simulink model "six_pulse_dstack_based_rectifier"  (R2026a)
settings: Solver=ode23tb  StopTime=simlength  FixedStep=Ts  MaxStep=Tc  EnableMultiTasking=on
values from neighbouring files (symbols this model uses):
  Csnubber = 0.1e-6    (= 1e-07)    [init_model.m]
  LFu_dc = 1.2e-3    (= 0.0012)    [init_model.m]
  Rgrading = 2.4e6    (= 2400000)    [init_model.m]
  RLFu_dc = 2e-4    (= 0.0002)    [init_model.m]
  Rsnubber = 1000    [init_model.m]
  Tc = Tcontrol_rect/4000    (= 5e-08)    [init_model.m]
  Tcontrol_rect = tPWM_RECT    (= 0.0002)    [init_model.m]
  Vnom_ac_adc = 400/sqrt(3)*sqrt(2)    [init_model.m]
  w_grid = f_grid*2*pi    (= 314.159265359)    [init_model.m]
undefined symbols (not defined in the file or in its folder): magnitude, rms
libraries: fl_lib x179, nesl_utility x129, diode_rr_lib x36, ee_lib x2
(part 1 of 5)
settings Model: Creator=LTNBDA  LastModifiedBy=d.bagnara
settings SolverCC: ZeroCrossControl=EnableAll  ZeroCrossAlgorithm=Adaptive  SolverResetMethod=Robust
settings DataIOCC: MaxDataPoints=1  SignalLoggingSaveFormat=ModelDataLogs
settings OptimizationCC: InitFltsAndDblsToZero=on  EfficientMapNaN2IntZero=off
settings DebuggingCC: SaveWithParameterizedLinksMsg=none  SignalResolutionControl=TryResolveAllWithWarning  MultiTaskDSMMsg=warning  MultiTaskCondExecSysMsg=none
settings HardwareCC: ProdBitPerLong=64.0  ProdHWDeviceType=Generic->64-bit Embedded Processor (LP64)  TargetBitPerPointer=64.0  TargetBitPerSizeT=64.0  TargetBitPerPtrDiffT=64.0  TargetLongLongMode=on  TargetIntDivRoundTo=Zero  TargetEndianess=LittleEndian  TargetWordSize=64.0  TargetHWDeviceType=MATLAB Host  ProdEqTarget=off
settings SFSimCC: SimCustomHeaderCode=|
  | #include "math_f.h"
  | #include "mavgflt.h"
  | #include "mavgflt_simulink.h"
  | #include "bemf_obsv.h"
  | #include "bemf_obsv_simulink.h"
  | #include "bemf_obsv_load_est.h"
  | #include "bemf_obsv_load_est_simulink.h"
  | #include "dqvector_pi.h"
  | #include "dqvector_pi_simulink.h"
  | #include "sv_pwm_simulink.h"
  | #include "sv_pwm.h"
  | #include "six_pulse_rect.h"
  | #include "twelve_pulse_rect.h"
  | #include "first_harmonic_tracker.h"
  | #include "first_harmonic_tracker_simulink.h"
  | #include "dqpll_thyr.h"
  | #include "dqpll_thyr_simulink.h"
  | #include "dqpll_grid.h"
  | #include "dqpll_grid_simulink.h"
settings SFSimCC: SimUserSources=|
  | "mavgflt_simulink.c"
  | "mavgflt.c"
  | "bemf_obsv_simulink.c"
  | "bemf_obsv.c"
  | "bemf_obsv_load_est_simulink.c"
  | "bemf_obsv_load_est.c"
  | "dqvector_pi.c"
  | "dqvector_pi_simulink.c"
  | "sv_pwm_simulink.c"
  | "sv_pwm.c"
  | "six_pulse_rect.c"
  | "twelve_pulse_rect.c"
  | "first_harmonic_tracker_simulink.c"
  | "first_harmonic_tracker.c"
  | "dqpll_thyr_simulink.c"
  | "dqpll_thyr.c"
  | "dqpll_grid_simulink.c"
  | "dqpll_grid.c"
settings SFSimCC: SimUserIncludeDirs=|
  | include
  | src
settings CodeAppCC: MaxIdLength=128.0
settings GRTTargetCC: CombineOutputUpdateFcns=off  GRTInterface=on
settings SimscapeCC: SimscapeNormalizeSystem=off  SimscapeNominalValues="[{\"value\":\"1\",\"unit\":\"A\"},{\"value\":\"1\",\"unit\":\"bar\"},{\"value\":\"1\",\"unit\":\"cm^2\"},{\"value\":\"1\",\"unit\":\"cm^3/s\"},{\"value\":\"1\",\"unit\":\"kJ/kg\"},{\"value\":\"1\",\"unit\":\"kW\"},{\"value\":\"1\",\"unit\":\"l\"},{\"value\":\"1\",\"unit\":\"N\"},{\"value\":\"1\",\"unit\":\"N*m\"},{\"value\":\"1\",\"unit\":\"V\"}]"  SimscapeLogType=none  SimscapeLogDataHistory=5000.0

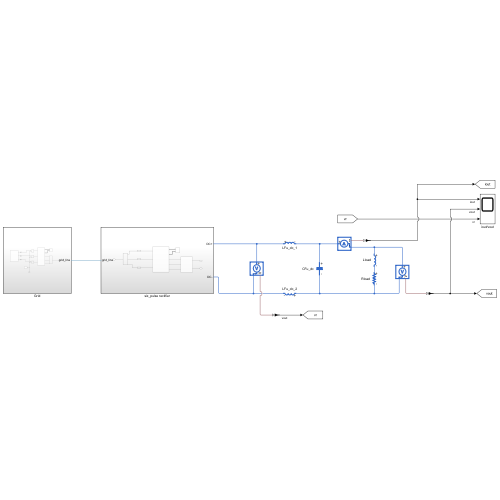
[thumbnail: Simulink's stored preview of the top-level diagram]
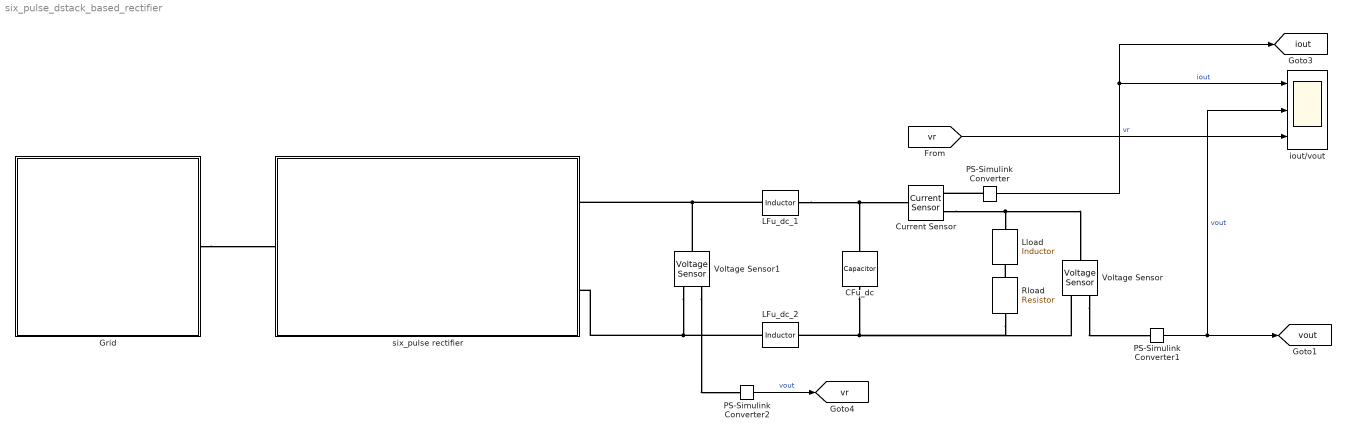
== system six_pulse_dstack_based_rectifier ==
  CFu_dc : fl_lib/Electrical/Electrical Elements/Capacitor  c=CFu_dc F  r=RCFu_dc Ohm  g=0 1/Ohm  i_specify=off  i_priority=None  i=0 A  i_nominal_specify=off  i_nominal_value=1  i_nominal_unit=A  v_specify=off  v_priority=None  v=0 V  v_nominal_specify=off  v_nominal_value=1  v_nominal_unit=V  vc_specify=off  vc_priority=High  vc=0 V  vc_nominal_specify=off  vc_nominal_value=1  vc_nominal_unit=V
  Current Sensor : fl_lib/Electrical/Electrical Sensors/Current Sensor
  Grid : Subsystem
  LFu_dc_1 : fl_lib/Electrical/Electrical Elements/Inductor  l=LFu_dc/2 H  r=RLFu_dc/2 Ohm  g=1e-9 1/Ohm  i_specify=off  i_priority=None  i=0 A  i_nominal_specify=off  i_nominal_value=1  i_nominal_unit=A  v_specify=off  v_priority=None  v=0 V  v_nominal_specify=off  v_nominal_value=1  v_nominal_unit=V  i_L_specify=off  i_L_priority=High  i_L=0 A  i_L_nominal_specify=off  i_L_nominal_value=1  i_L_nominal_unit=A
  LFu_dc_2 : fl_lib/Electrical/Electrical Elements/Inductor  l=LFu_dc/2 H  r=RLFu_dc/2 Ohm  g=1e-9 1/Ohm  i_specify=off  i_priority=None  i=0 A  i_nominal_specify=off  i_nominal_value=1  i_nominal_unit=A  v_specify=off  v_priority=None  v=0 V  v_nominal_specify=off  v_nominal_value=1  v_nominal_unit=V  i_L_specify=off  i_L_priority=High  i_L=0 A  i_L_nominal_specify=off  i_L_nominal_value=1  i_L_nominal_unit=A
  Lload : fl_lib/Electrical/Electrical Elements/Inductor  l=Lload H  r=0 Ohm  g=1e-9 1/Ohm  i_specify=off  i_priority=None  i=0 A  i_nominal_specify=off  i_nominal_value=1  i_nominal_unit=A  v_specify=off  v_priority=None  v=0 V  v_nominal_specify=off  v_nominal_value=1  v_nominal_unit=V  i_L_specify=off  i_L_priority=High  i_L=0 A  i_L_nominal_specify=off  i_L_nominal_value=1  i_L_nominal_unit=A
  PS-Simulink Converter : nesl_utility/PS-Simulink Converter  PhysicalDomain=network_engine_domain  SubClassName=ps_output  LeftPortType=input  RightPortType=output  PseudoPeriodic=off  Frequencies=[]  VectorFormat=1-D array  Unit=A  AffineConversion=off
  PS-Simulink Converter1 : nesl_utility/PS-Simulink Converter  PhysicalDomain=network_engine_domain  SubClassName=ps_output  LeftPortType=input  RightPortType=output  PseudoPeriodic=off  Frequencies=[]  VectorFormat=1-D array  Unit=V  AffineConversion=on
  PS-Simulink Converter2 : nesl_utility/PS-Simulink Converter  PhysicalDomain=network_engine_domain  SubClassName=ps_output  LeftPortType=input  RightPortType=output  PseudoPeriodic=off  Frequencies=[]  VectorFormat=1-D array  Unit=V  AffineConversion=on
  Rload : fl_lib/Electrical/Electrical Elements/Resistor  R=(13.8e3*1.35)^2/1e6 Ohm  i_specify=off  i_priority=None  i=0 A  i_nominal_specify=off  i_nominal_value=1  i_nominal_unit=A  v_specify=off  v_priority=None  v=0 V  v_nominal_specify=off  v_nominal_value=1  v_nominal_unit=V
  Voltage Sensor : fl_lib/Electrical/Electrical Sensors/Voltage Sensor
  Voltage Sensor1 : fl_lib/Electrical/Electrical Sensors/Voltage Sensor
  iout/vout : Scope  NumInputPorts=3
      settings: ActiveDisplayYMinimum=54.4311221075266  ActiveDisplayYMaximum=54.825714064717985  DataLoggingVariableName=ScopeData10
  six_pulse rectifier : Subsystem
  tag scope: iout=global, vout=global, vr=global
  wires:
  PS-Simulink Converter/1 -> [iout], iout/vout/1  "iout"
  PS-Simulink Converter1/1 -> [vout], iout/vout/2  "vout"
  PS-Simulink Converter2/1 -> [vr]  "vout"
  [vr] -> iout/vout/3  "vr"
  connections:
  LFu_dc_1/RConn1 -- CFu_dc/LConn1 -- Current Sensor/LConn1
  CFu_dc/RConn1 -- Voltage Sensor/RConn2 -- Rload/RConn1 -- LFu_dc_2/LConn1
  LFu_dc_2/RConn1 -- Voltage Sensor1/RConn2 -- six_pulse rectifier/RConn2
  LFu_dc_1/LConn1 -- six_pulse rectifier/RConn1 -- Voltage Sensor1/LConn1
  Rload/LConn1 -- Lload/RConn1
  PS-Simulink Converter/LConn1 -- Current Sensor/RConn1
  Current Sensor/RConn2 -- Voltage Sensor/LConn1 -- Lload/LConn1
  Voltage Sensor/RConn1 -- PS-Simulink Converter1/LConn1
  Voltage Sensor1/RConn1 -- PS-Simulink Converter2/LConn1
  Grid/RConn1 -- six_pulse rectifier/LConn1

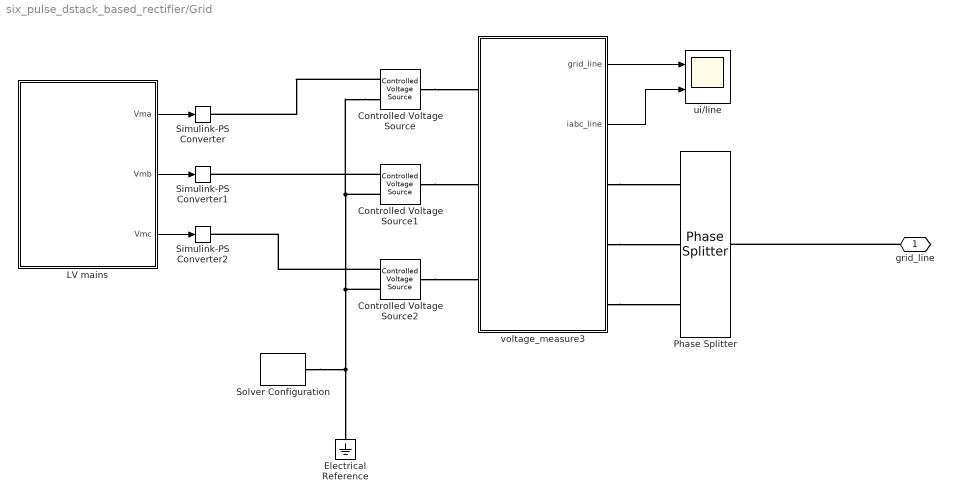
== system six_pulse_dstack_based_rectifier/Grid ==
  Controlled Voltage Source : fl_lib/Electrical/Electrical Sources/Controlled Voltage Source
  Controlled Voltage Source1 : fl_lib/Electrical/Electrical Sources/Controlled Voltage Source
  Controlled Voltage Source2 : fl_lib/Electrical/Electrical Sources/Controlled Voltage Source
  Electrical Reference : fl_lib/Electrical/Electrical Elements/Electrical Reference
  LV mains : Subsystem
  Phase Splitter : ee_lib/Connectors & References/Phase Splitter
  Simulink-PS Converter : nesl_utility/Simulink-PS Converter  PhysicalDomain=network_engine_domain  SubClassName=ps_input  LeftPortType=input  RightPortType=output  PseudoPeriodic=off  Frequencies=[]  NoiseDistribution=none  NoiseParameters=[]  Unit=V  AffineConversion=on  FilteringAndDerivatives=provide  SimscapeFilterOrder=1  InputFilterTimeConstant=0.001  UdotUserProvided=0
  Simulink-PS Converter1 : nesl_utility/Simulink-PS Converter  PhysicalDomain=network_engine_domain  SubClassName=ps_input  LeftPortType=input  RightPortType=output  PseudoPeriodic=off  Frequencies=[]  NoiseDistribution=none  NoiseParameters=[]  Unit=V  AffineConversion=on  FilteringAndDerivatives=provide  SimscapeFilterOrder=1  InputFilterTimeConstant=0.001  UdotUserProvided=0
  Simulink-PS Converter2 : nesl_utility/Simulink-PS Converter  PhysicalDomain=network_engine_domain  SubClassName=ps_input  LeftPortType=input  RightPortType=output  PseudoPeriodic=off  Frequencies=[]  NoiseDistribution=none  NoiseParameters=[]  Unit=V  AffineConversion=on  FilteringAndDerivatives=provide  SimscapeFilterOrder=1  InputFilterTimeConstant=0.001  UdotUserProvided=0
  Solver Configuration : nesl_utility/Solver Configuration  PhysicalDomain=network_engine_domain  SubClassName=solver  LeftPortType=input  RightPortType=generic  Tones=[]  Harmonics=[]  SimulateNoise=off  Profile=off  UseLocalSampling=off  EnableSwitchedLinearOptims=on  FrequencyDomain=off  UseCCode=off  RelTol=0.001  AbsTol=1e-06  MinStep=1e-09  ToWorkspace=off  RevertToSquareIcSolve=off  NumHomotopyIterations=100  PhasorMode=off  PhasorModeNumHarmonics=1  ConsistencySolver=NEWTON_FTOL  CanonicalOrdering=UNORDERED  OptimizeIntermediates=UNOPTIMIZED  IndexReductionMethod=DerivativeReplacement  DoDC=on  ResidualTolerance=1e-4  ConsistencyTolSource=GLOBAL  ConsistencyAbsTol=0.001  ConsistencyRelTol=0.001  ConsistencyTolFactor=0.001  UseLocalSolver=on  LocalSolverChoice=NE_TRAPEZOIDAL_ADVANCER  ResolveIndetEquations=on  FunctionEvalNumThread=1  LocalSolverSampleTime=Tc  DoFixedCost=on  MaxNonlinIter=5  MaxModeIter=2  ComputeImpulses=off  ImpulseIterations=2  LinearAlgebra=auto  LinearAlgebraNumThread=0  EquationFormulation=NE_TIME_EF  DelaysMemoryBudget=1024  AutomaticFiltering=on  FilteringTimeConstant=0.001  PartitionStorageMethod=AS_NEEDED  PartitionMemoryBudget=1024  PartitionMethod=ROBUST  MultibodyUseLocalSolver=off  MultibodyLocalSolverChoice=ODE1  MultibodyLocalSolverSampleTime=0.001
  ui/line : Scope  NumInputPorts=2
      settings: SampleTime=Tcontrol_rect  ActiveDisplayYMinimum=-1.25  ActiveDisplayYMaximum=1.25
  voltage_measure3 : Subsystem
  grid_line : PMIOPort  Side=Right
  wires:
  voltage_measure3/2(iabc_line) -> ui/line/2
  LV mains/1(Vma) -> Simulink-PS Converter/1
  LV mains/3(Vmc) -> Simulink-PS Converter2/1
  LV mains/2(Vmb) -> Simulink-PS Converter1/1
  voltage_measure3/1(grid_line) -> ui/line/1
  connections:
  Controlled Voltage Source1/LConn1 -- voltage_measure3/LConn2
  grid_line/RConn1 -- Phase Splitter/LConn1
  Controlled Voltage Source/RConn1 -- Simulink-PS Converter/RConn1
  Controlled Voltage Source/RConn2 -- Controlled Voltage Source1/RConn2 -- Controlled Voltage Source2/RConn2 -- Solver Configuration/RConn1 -- Electrical Reference/LConn1
  voltage_measure3/RConn2 -- Phase Splitter/RConn2
  Controlled Voltage Source2/LConn1 -- voltage_measure3/LConn3
  voltage_measure3/RConn3 -- Phase Splitter/RConn3
  Controlled Voltage Source1/RConn1 -- Simulink-PS Converter1/RConn1
  Controlled Voltage Source2/RConn1 -- Simulink-PS Converter2/RConn1
  Controlled Voltage Source/LConn1 -- voltage_measure3/LConn1
  voltage_measure3/RConn1 -- Phase Splitter/RConn1

== system six_pulse_dstack_based_rectifier/six_pulse rectifier ==
  BR2 : Subsystem
  Lgrid_U : fl_lib/Electrical/Electrical Elements/Inductor  l=31e-3 H  r=0 Ohm  g=1e-9 1/Ohm  i_specify=off  i_priority=None  i=0 A  i_nominal_specify=off  i_nominal_value=1  i_nominal_unit=A  v_specify=off  v_priority=None  v=0 V  v_nominal_specify=off  v_nominal_value=1  v_nominal_unit=V  i_L_specify=off  i_L_priority=High  i_L=0 A  i_L_nominal_specify=off  i_L_nominal_value=1  i_L_nominal_unit=A
  Lgrid_V : fl_lib/Electrical/Electrical Elements/Inductor  l=31e-3 H  r=0 Ohm  g=1e-9 1/Ohm  i_specify=off  i_priority=None  i=0 A  i_nominal_specify=off  i_nominal_value=1  i_nominal_unit=A  v_specify=off  v_priority=None  v=0 V  v_nominal_specify=off  v_nominal_value=1  v_nominal_unit=V  i_L_specify=off  i_L_priority=High  i_L=0 A  i_L_nominal_specify=off  i_L_nominal_value=1  i_L_nominal_unit=A
  Lgrid_W : fl_lib/Electrical/Electrical Elements/Inductor  l=31e-3 H  r=0 Ohm  g=1e-9 1/Ohm  i_specify=off  i_priority=None  i=0 A  i_nominal_specify=off  i_nominal_value=1  i_nominal_unit=A  v_specify=off  v_priority=None  v=0 V  v_nominal_specify=off  v_nominal_value=1  v_nominal_unit=V  i_L_specify=off  i_L_priority=High  i_L=0 A  i_L_nominal_specify=off  i_L_nominal_value=1  i_L_nominal_unit=A
  Phase Splitter2 : ee_lib/Connectors & References/Phase Splitter
  ui/grid : Scope  NumInputPorts=2
      settings: ActiveDisplayYMinimum=-46.896074870279  ActiveDisplayYMaximum=64.47147383027982
  voltage_measure2 : Subsystem
  DC+ : PMIOPort  Side=Right
  grid_line : PMIOPort  Port=2  Side=Left
  DC- : PMIOPort  Port=3  Side=Right
  wires:
  voltage_measure2/1(vabc_grid) -> ui/grid/1
  voltage_measure2/2(iabc_grid) -> ui/grid/2
  connections:
  voltage_measure2/RConn1 -- BR2/RConn1
  grid_line/RConn1 -- Phase Splitter2/LConn1
  BR2/LConn2 -- DC-/RConn1
  voltage_measure2/RConn3 -- BR2/RConn3
  Lgrid_U/RConn1 -- voltage_measure2/LConn1
  voltage_measure2/RConn2 -- BR2/RConn2
  BR2/LConn1 -- DC+/RConn1
  Phase Splitter2/RConn1 -- Lgrid_U/LConn1
  Lgrid_V/RConn1 -- voltage_measure2/LConn2
  Lgrid_V/LConn1 -- Phase Splitter2/RConn2
  Lgrid_W/LConn1 -- Phase Splitter2/RConn3
  Lgrid_W/RConn1 -- voltage_measure2/LConn3

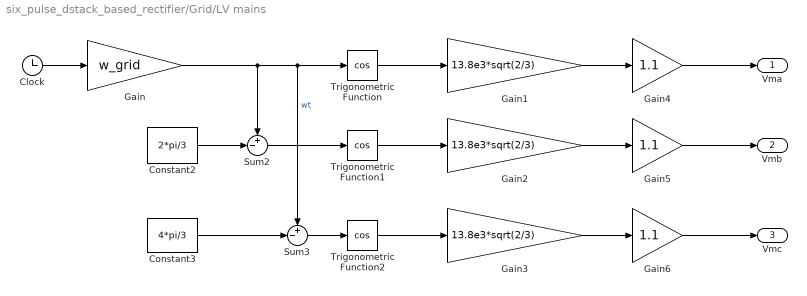
== system six_pulse_dstack_based_rectifier/Grid/LV mains ==
  Clock : Clock
  Constant2 : Constant  Value=2*pi/3
  Constant3 : Constant  Value=4*pi/3
  Gain : Gain  Gain=w_grid
  Gain1 : Gain  Gain=13.8e3*sqrt(2/3)
  Gain2 : Gain  Gain=13.8e3*sqrt(2/3)
  Gain3 : Gain  Gain=13.8e3*sqrt(2/3)
  Gain4 : Gain  Gain=1.1
  Gain5 : Gain  Gain=1.1
  Gain6 : Gain  Gain=1.1
  Sum2 : Sum  Inputs=+-|
  Sum3 : Sum  Inputs=+-|
  Trigonometric Function : Trigonometry  Operator=cos
  Trigonometric Function1 : Trigonometry  Operator=cos
  Trigonometric Function2 : Trigonometry  Operator=cos
  Vma : Outport
  Vmb : Outport  Port=2
  Vmc : Outport  Port=3
  wires:
  Trigonometric Function/1 -> Gain1/1
  Constant2/1 -> Sum2/2
  Sum2/1 -> Trigonometric Function1/1
  Constant3/1 -> Sum3/2
  Sum3/1 -> Trigonometric Function2/1
  Clock/1 -> Gain/1
  Gain/1 -> Sum3/1, Trigonometric Function/1, Sum2/1  "wt"
  Trigonometric Function1/1 -> Gain2/1
  Trigonometric Function2/1 -> Gain3/1
  Gain1/1 -> Gain4/1
  Gain2/1 -> Gain5/1
  Gain3/1 -> Gain6/1
  Gain4/1 -> Vma/1
  Gain5/1 -> Vmb/1
  Gain6/1 -> Vmc/1

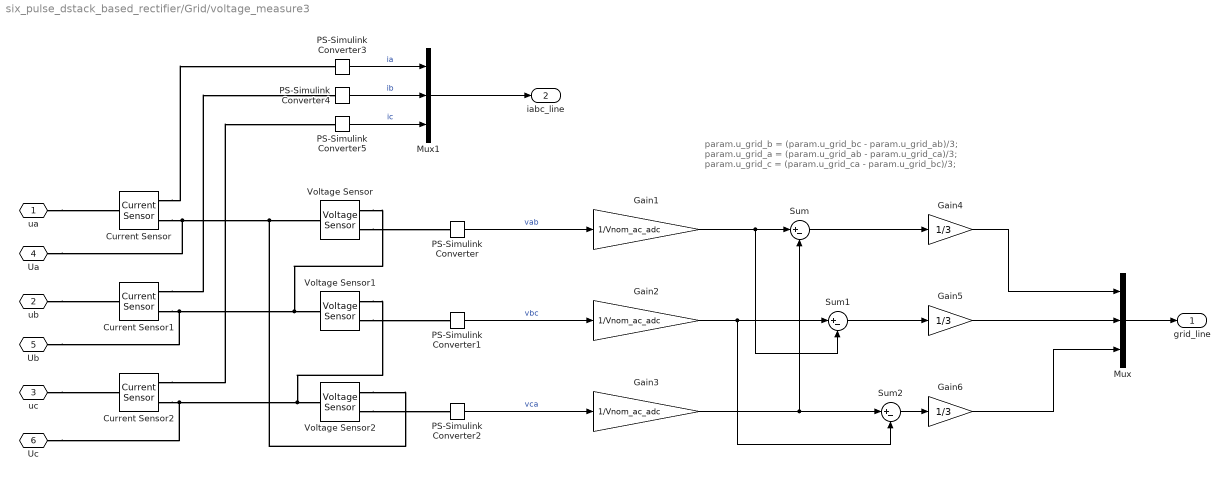
== system six_pulse_dstack_based_rectifier/Grid/voltage_measure3 ==
  note: param.u_grid_b = (param.u_grid_bc - param.u_grid_ab)/3;
      | 	param.u_grid_a = (param.u_grid_ab - param.u_grid_ca)/3;
      | 	param.u_grid_c = (param.u_grid_ca - param.u_grid_bc)/3;
  Current Sensor : fl_lib/Electrical/Electrical Sensors/Current Sensor
  Current Sensor1 : fl_lib/Electrical/Electrical Sensors/Current Sensor
  Current Sensor2 : fl_lib/Electrical/Electrical Sensors/Current Sensor
  Gain1 : Gain  Gain=1/Vnom_ac_adc
  Gain2 : Gain  Gain=1/Vnom_ac_adc
  Gain3 : Gain  Gain=1/Vnom_ac_adc
  Gain4 : Gain  Gain=1/3
  Gain5 : Gain  Gain=1/3
  Gain6 : Gain  Gain=1/3
  Mux : Mux  Inputs=3
  Mux1 : Mux  Inputs=3
  PS-Simulink Converter : nesl_utility/PS-Simulink Converter  PhysicalDomain=network_engine_domain  SubClassName=ps_output  LeftPortType=input  RightPortType=output  PseudoPeriodic=off  Frequencies=[]  VectorFormat=1-D array  Unit=inherit  AffineConversion=off
  PS-Simulink Converter1 : nesl_utility/PS-Simulink Converter  PhysicalDomain=network_engine_domain  SubClassName=ps_output  LeftPortType=input  RightPortType=output  PseudoPeriodic=off  Frequencies=[]  VectorFormat=1-D array  Unit=inherit  AffineConversion=off
  PS-Simulink Converter2 : nesl_utility/PS-Simulink Converter  PhysicalDomain=network_engine_domain  SubClassName=ps_output  LeftPortType=input  RightPortType=output  PseudoPeriodic=off  Frequencies=[]  VectorFormat=1-D array  Unit=inherit  AffineConversion=off
  PS-Simulink Converter3 : nesl_utility/PS-Simulink Converter  PhysicalDomain=network_engine_domain  SubClassName=ps_output  LeftPortType=input  RightPortType=output  PseudoPeriodic=off  Frequencies=[]  VectorFormat=1-D array  Unit=A  AffineConversion=off
  PS-Simulink Converter4 : nesl_utility/PS-Simulink Converter  PhysicalDomain=network_engine_domain  SubClassName=ps_output  LeftPortType=input  RightPortType=output  PseudoPeriodic=off  Frequencies=[]  VectorFormat=1-D array  Unit=A  AffineConversion=off
  PS-Simulink Converter5 : nesl_utility/PS-Simulink Converter  PhysicalDomain=network_engine_domain  SubClassName=ps_output  LeftPortType=input  RightPortType=output  PseudoPeriodic=off  Frequencies=[]  VectorFormat=1-D array  Unit=A  AffineConversion=off
  Sum : Sum  Inputs=|+-
  Sum1 : Sum  Inputs=|+-
  Sum2 : Sum  Inputs=|+-
  Voltage Sensor : fl_lib/Electrical/Electrical Sensors/Voltage Sensor
  Voltage Sensor1 : fl_lib/Electrical/Electrical Sensors/Voltage Sensor
  Voltage Sensor2 : fl_lib/Electrical/Electrical Sensors/Voltage Sensor
  ua : PMIOPort  Side=Left
  ub : PMIOPort  Port=2  Side=Left
  uc : PMIOPort  Port=3  Side=Left
  Ua : PMIOPort  Port=4  Side=Right
  Ub : PMIOPort  Port=5  Side=Right
  Uc : PMIOPort  Port=6  Side=Right
  grid_line : Outport
  iabc_line : Outport  Port=2
  wires:
  PS-Simulink Converter5/1 -> Mux1/3  "ic"
  PS-Simulink Converter3/1 -> Mux1/1  "ia"
  PS-Simulink Converter4/1 -> Mux1/2  "ib"
  Mux1/1 -> iabc_line/1
  Gain6/1 -> Mux/3
  Gain5/1 -> Mux/2
  Gain4/1 -> Mux/1
  Gain2/1 -> Sum1/1, Sum2/2
  Sum2/1 -> Gain6/1
  Sum1/1 -> Gain5/1
  Sum/1 -> Gain4/1
  Gain3/1 -> Sum/2, Sum2/1
  Gain1/1 -> Sum/1, Sum1/2
  Mux/1 -> grid_line/1
  PS-Simulink Converter/1 -> Gain1/1  "vab"
  PS-Simulink Converter2/1 -> Gain3/1  "vca"
  PS-Simulink Converter1/1 -> Gain2/1  "vbc"
  connections:
  Current Sensor2/RConn1 -- PS-Simulink Converter5/LConn1
  Current Sensor1/RConn1 -- PS-Simulink Converter4/LConn1
  Current Sensor/RConn1 -- PS-Simulink Converter3/LConn1
  uc/RConn1 -- Current Sensor2/LConn1
  ub/RConn1 -- Current Sensor1/LConn1
  ua/RConn1 -- Current Sensor/LConn1
  Voltage Sensor1/RConn1 -- PS-Simulink Converter1/LConn1
  Uc/RConn1 -- Current Sensor2/RConn2 -- Voltage Sensor1/RConn2 -- Voltage Sensor2/LConn1
  Voltage Sensor2/RConn1 -- PS-Simulink Converter2/LConn1
  Voltage Sensor/RConn1 -- PS-Simulink Converter/LConn1
  Ua/RConn1 -- Current Sensor/RConn2 -- Voltage Sensor2/RConn2 -- Voltage Sensor/LConn1
  Ub/RConn1 -- Current Sensor1/RConn2 -- Voltage Sensor/RConn2 -- Voltage Sensor1/LConn1

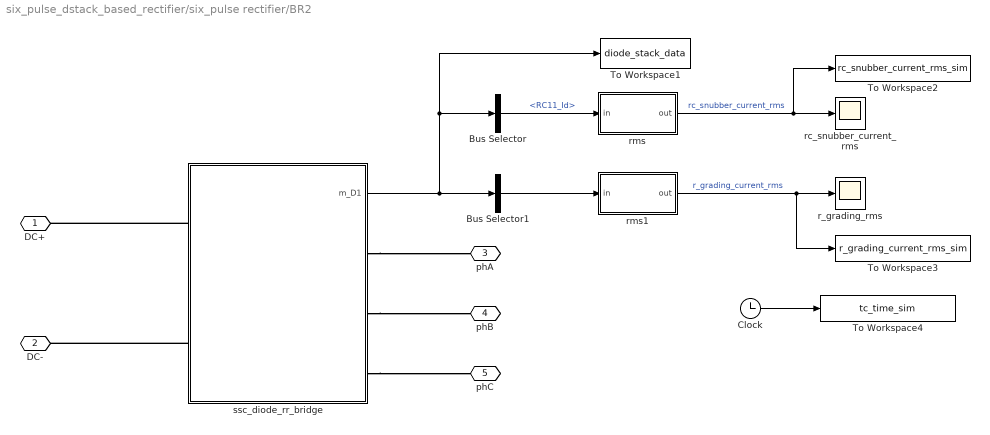
== system six_pulse_dstack_based_rectifier/six_pulse rectifier/BR2 ==
  Bus Selector : BusSelector  OutputSignals=signal1.RC11_Id
  Bus Selector1 : BusSelector  OutputSignals=signal4.Rg11_I  OutputAsBus=on
  Clock : Clock
  To Workspace1 : ToWorkspace  VariableName=diode_stack_data  SaveFormat=Structure With Time  SampleTime=Tc
      settings: MaxDataPoints=Nc
  To Workspace2 : ToWorkspace  VariableName=rc_snubber_current_rms_sim  SaveFormat=Structure With Time  SampleTime=Tc
      settings: MaxDataPoints=Nc
  To Workspace3 : ToWorkspace  VariableName=r_grading_current_rms_sim  SaveFormat=Structure With Time  SampleTime=Tc
      settings: MaxDataPoints=Nc
  To Workspace4 : ToWorkspace  VariableName=tc_time_sim  SaveFormat=Structure With Time  SampleTime=Tc
      settings: MaxDataPoints=Nc
  r_grading_rms : Scope
      settings: ActiveDisplayYMinimum=-0.00012535770795036924  ActiveDisplayYMaximum=0.0011282275135877779
  rc_snubber_current_rms : Scope
      settings: ActiveDisplayYMinimum=-0.017079152210377417  ActiveDisplayYMaximum=0.15371236989339679  DataLoggingVariableName=ScopeData8
  rms : Subsystem
  rms1 : Subsystem
  ssc_diode_rr_bridge : Subsystem  mask{Vf_m=1.12, Ron_m=0.29e-3, Goff_m=1e-5, forward_voltage_threshold_m=50, Vgt_m=1.2, latching_current_m=250e-3, holding_current_m=75e-3, carrier_lifetime_m=100e-6, charge_cross_time_constant_m=190e-6, residual_charge_threshold_m=1e-6, circuit_commutated_turn_off_time_m=800e-6, t_firing_strobe_m=Tcontrol_rect, Rsnubber_m=Rsnubber, Csnubber_m=Csnubber, Rgrading_m=Rgrading}
      mask prompts: Vf_m "Vt [V]"; Ron_m "rt [Ohm]"; Goff_m "Goff [1/Ohm]"; forward_voltage_threshold_m "Voltage Retrigger Threshold [V]"; Vgt_m "Vth [V]"; latching_current_m "latching current [A]"; holding_current_m "holding current [A]"; carrier_lifetime_m "carrier lifetime [s]"; charge_cross_time_constant_m "charge extraction time constant [s]"; residual_charge_threshold_m "residual charge threshold [C]"; circuit_commutated_turn_off_time_m "circuit commutated turn off time [s]"; t_firing_strobe_m "t_firing_strobe [s]"; Rsnubber_m "Rsnubber [Ohm]"; Csnubber_m "Csnubber [F]"; Rgrading_m "Rgrading [Ohm]"
  DC+ : PMIOPort  Side=Left
  DC- : PMIOPort  Port=2  Side=Left
  phA : PMIOPort  Port=3  Side=Right
  phB : PMIOPort  Port=4  Side=Right
  phC : PMIOPort  Port=5  Side=Right
  wires:
  rms/1(out) -> To Workspace2/1, rc_snubber_current_rms/1  "rc_snubber_current_rms"
  ssc_diode_rr_bridge/1(m_D1) -> Bus Selector/1, To Workspace1/1, Bus Selector1/1
  Bus Selector/1 -> rms/1(in)  "<RC11_Id>"
  Bus Selector1/1 -> rms1/1(in)
  rms1/1(out) -> To Workspace3/1, r_grading_rms/1  "r_grading_current_rms"
  Clock/1 -> To Workspace4/1
  connections:
  ssc_diode_rr_bridge/LConn1 -- DC+/RConn1
  ssc_diode_rr_bridge/LConn2 -- DC-/RConn1
  ssc_diode_rr_bridge/RConn1 -- phA/RConn1
  ssc_diode_rr_bridge/RConn2 -- phB/RConn1
  ssc_diode_rr_bridge/RConn3 -- phC/RConn1

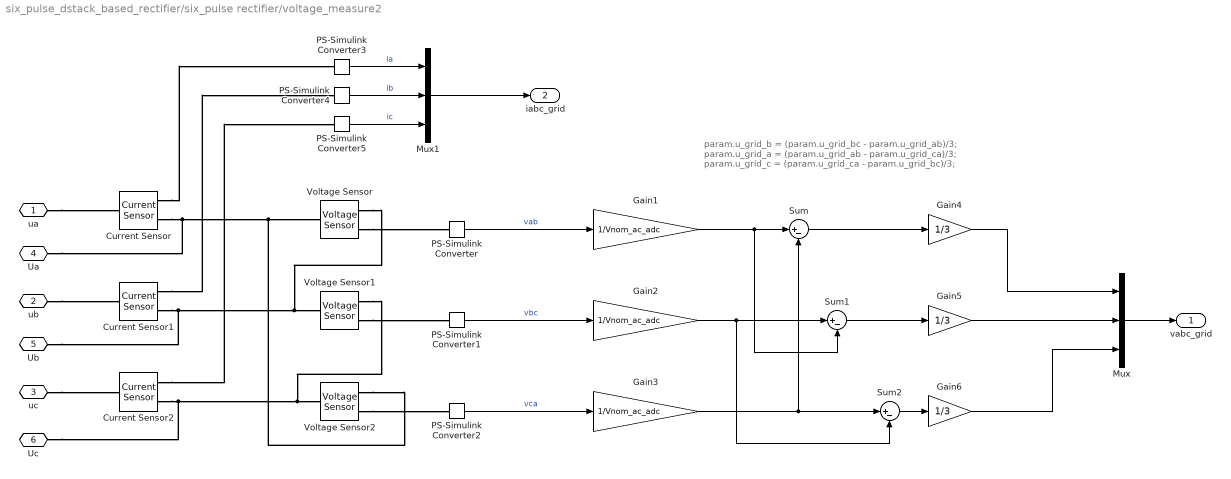
== system six_pulse_dstack_based_rectifier/six_pulse rectifier/voltage_measure2 ==
  note: param.u_grid_b = (param.u_grid_bc - param.u_grid_ab)/3;
      | 	param.u_grid_a = (param.u_grid_ab - param.u_grid_ca)/3;
      | 	param.u_grid_c = (param.u_grid_ca - param.u_grid_bc)/3;
  Current Sensor : fl_lib/Electrical/Electrical Sensors/Current Sensor
  Current Sensor1 : fl_lib/Electrical/Electrical Sensors/Current Sensor
  Current Sensor2 : fl_lib/Electrical/Electrical Sensors/Current Sensor
  Gain1 : Gain  Gain=1/Vnom_ac_adc
  Gain2 : Gain  Gain=1/Vnom_ac_adc
  Gain3 : Gain  Gain=1/Vnom_ac_adc
  Gain4 : Gain  Gain=1/3
  Gain5 : Gain  Gain=1/3
  Gain6 : Gain  Gain=1/3
  Mux : Mux  Inputs=3
  Mux1 : Mux  Inputs=3
  PS-Simulink Converter : nesl_utility/PS-Simulink Converter  PhysicalDomain=network_engine_domain  SubClassName=ps_output  LeftPortType=input  RightPortType=output  PseudoPeriodic=off  Frequencies=[]  VectorFormat=1-D array  Unit=inherit  AffineConversion=off
  PS-Simulink Converter1 : nesl_utility/PS-Simulink Converter  PhysicalDomain=network_engine_domain  SubClassName=ps_output  LeftPortType=input  RightPortType=output  PseudoPeriodic=off  Frequencies=[]  VectorFormat=1-D array  Unit=inherit  AffineConversion=off
  PS-Simulink Converter2 : nesl_utility/PS-Simulink Converter  PhysicalDomain=network_engine_domain  SubClassName=ps_output  LeftPortType=input  RightPortType=output  PseudoPeriodic=off  Frequencies=[]  VectorFormat=1-D array  Unit=inherit  AffineConversion=off
  PS-Simulink Converter3 : nesl_utility/PS-Simulink Converter  PhysicalDomain=network_engine_domain  SubClassName=ps_output  LeftPortType=input  RightPortType=output  PseudoPeriodic=off  Frequencies=[]  VectorFormat=1-D array  Unit=A  AffineConversion=off
  PS-Simulink Converter4 : nesl_utility/PS-Simulink Converter  PhysicalDomain=network_engine_domain  SubClassName=ps_output  LeftPortType=input  RightPortType=output  PseudoPeriodic=off  Frequencies=[]  VectorFormat=1-D array  Unit=A  AffineConversion=off
  PS-Simulink Converter5 : nesl_utility/PS-Simulink Converter  PhysicalDomain=network_engine_domain  SubClassName=ps_output  LeftPortType=input  RightPortType=output  PseudoPeriodic=off  Frequencies=[]  VectorFormat=1-D array  Unit=A  AffineConversion=off
  Sum : Sum  Inputs=|+-
  Sum1 : Sum  Inputs=|+-
  Sum2 : Sum  Inputs=|+-
  Voltage Sensor : fl_lib/Electrical/Electrical Sensors/Voltage Sensor
  Voltage Sensor1 : fl_lib/Electrical/Electrical Sensors/Voltage Sensor
  Voltage Sensor2 : fl_lib/Electrical/Electrical Sensors/Voltage Sensor
  ua : PMIOPort  Side=Left
  ub : PMIOPort  Port=2  Side=Left
  uc : PMIOPort  Port=3  Side=Left
  Ua : PMIOPort  Port=4  Side=Right
  Ub : PMIOPort  Port=5  Side=Right
  Uc : PMIOPort  Port=6  Side=Right
  vabc_grid : Outport
  iabc_grid : Outport  Port=2
  wires:
  PS-Simulink Converter1/1 -> Gain2/1  "vbc"
  PS-Simulink Converter2/1 -> Gain3/1  "vca"
  PS-Simulink Converter/1 -> Gain1/1  "vab"
  Mux/1 -> vabc_grid/1
  Gain1/1 -> Sum1/2, Sum/1
  Gain3/1 -> Sum2/1, Sum/2
  Sum/1 -> Gain4/1
  Sum1/1 -> Gain5/1
  Sum2/1 -> Gain6/1
  Gain2/1 -> Sum2/2, Sum1/1
  Gain4/1 -> Mux/1
  Gain5/1 -> Mux/2
  Gain6/1 -> Mux/3
  Mux1/1 -> iabc_grid/1
  PS-Simulink Converter4/1 -> Mux1/2  "ib"
  PS-Simulink Converter3/1 -> Mux1/1  "ia"
  PS-Simulink Converter5/1 -> Mux1/3  "ic"
  connections:
  Ub/RConn1 -- Current Sensor1/RConn2 -- Voltage Sensor/RConn2 -- Voltage Sensor1/LConn1
  Ua/RConn1 -- Current Sensor/RConn2 -- Voltage Sensor2/RConn2 -- Voltage Sensor/LConn1
  Voltage Sensor/RConn1 -- PS-Simulink Converter/LConn1
  Voltage Sensor2/RConn1 -- PS-Simulink Converter2/LConn1
  Uc/RConn1 -- Current Sensor2/RConn2 -- Voltage Sensor1/RConn2 -- Voltage Sensor2/LConn1
  Voltage Sensor1/RConn1 -- PS-Simulink Converter1/LConn1
  ua/RConn1 -- Current Sensor/LConn1
  ub/RConn1 -- Current Sensor1/LConn1
  uc/RConn1 -- Current Sensor2/LConn1
  Current Sensor/RConn1 -- PS-Simulink Converter3/LConn1
  Current Sensor1/RConn1 -- PS-Simulink Converter4/LConn1
  Current Sensor2/RConn1 -- PS-Simulink Converter5/LConn1

== system six_pulse_dstack_based_rectifier/six_pulse rectifier/BR2/rms ==
  in : Inport
  Gain : Gain  Gain=rms.n1-1
  Gain1 : Gain  Gain=1/rms.n1
  Math Function : Math  Operator=magnitude^2  SignedPower=on
  Sqrt : Sqrt
  Sum : Sum  Inputs=|++
  Unit Delay : UnitDelay  SampleTime=Tc
  out : Outport  VectorParamsAs1DForOutWhenUnconnected=off
  wires:
  in/1 -> Math Function/1
  Sum/1 -> Gain1/1
  Gain1/1 -> Sqrt/1, Unit Delay/1
  Unit Delay/1 -> Gain/1
  Math Function/1 -> Sum/1
  Sqrt/1 -> out/1
  Gain/1 -> Sum/2

== system six_pulse_dstack_based_rectifier/six_pulse rectifier/BR2/rms1 ==
  in : Inport
  Gain : Gain  Gain=rms.n1-1
  Gain1 : Gain  Gain=1/rms.n1
  Math Function : Math  Operator=magnitude^2  SignedPower=on
  Sqrt : Sqrt
  Sum : Sum  Inputs=|++
  Unit Delay : UnitDelay  SampleTime=Tc
  out : Outport  VectorParamsAs1DForOutWhenUnconnected=off
  wires:
  Gain/1 -> Sum/2
  Sqrt/1 -> out/1
  Math Function/1 -> Sum/1
  Unit Delay/1 -> Gain/1
  Gain1/1 -> Unit Delay/1, Sqrt/1
  Sum/1 -> Gain1/1
  in/1 -> Math Function/1

== system six_pulse_dstack_based_rectifier/six_pulse rectifier/BR2/ssc_diode_rr_bridge ==
  D1 : Subsystem
      settings: PortSchema="{\"entries\":[{\"content\":{\"sides\":[{\"content\":{\"connectorIds\":[\"LConn1\"]},\"type\":\"ConnectorPlacement.EquallySpacedRectSide\",\"uuid\":\"eb17bf97-c788-4c08-b023-8c0a1c3fb797\"},{\"content\":{\"connectorIds\":[\"RConn1\"],\"side\":\"RIGHT\"},\"type\":\"ConnectorPlacement.EquallySpacedRectSide\",\"uuid\":\"91e808db-0093-47a9-9188-f8caa3465017\"},{\"content\":{\"connectorIds\":[\"Out1\"],\"side\":\"TOP\"},\"type\":\"ConnectorPlacement.EquallySpacedRectSide\",\"uuid\":\"c8f1b688-6876-4a25-941d-460dbd5f524f\"}]},\"type\":\"ConnectorPlacement.EquallySpacedConnector\",\"uuid\":\"ee394044-67a1-441d-b622-768cddf1663c\"}],\"packageUris\":[\"http://schema.mathworks.com/mf0/Connector/R2020b\"],\"version\":\"1.0\"}"
  D2 : Subsystem
      settings: PortSchema="{\"entries\":[{\"content\":{\"sides\":[{\"content\":{\"connectorIds\":[\"LConn1\"]},\"type\":\"ConnectorPlacement.EquallySpacedRectSide\",\"uuid\":\"eb17bf97-c788-4c08-b023-8c0a1c3fb797\"},{\"content\":{\"connectorIds\":[\"RConn1\"],\"side\":\"RIGHT\"},\"type\":\"ConnectorPlacement.EquallySpacedRectSide\",\"uuid\":\"91e808db-0093-47a9-9188-f8caa3465017\"},{\"content\":{\"connectorIds\":[\"Out1\"],\"side\":\"TOP\"},\"type\":\"ConnectorPlacement.EquallySpacedRectSide\",\"uuid\":\"c8f1b688-6876-4a25-941d-460dbd5f524f\"}]},\"type\":\"ConnectorPlacement.EquallySpacedConnector\",\"uuid\":\"ee394044-67a1-441d-b622-768cddf1663c\"}],\"packageUris\":[\"http://schema.mathworks.com/mf0/Connector/R2020b\"],\"version\":\"1.0\"}"
  D3 : Subsystem
      settings: PortSchema="{\"entries\":[{\"content\":{\"sides\":[{\"content\":{\"connectorIds\":[\"LConn1\"]},\"type\":\"ConnectorPlacement.EquallySpacedRectSide\",\"uuid\":\"eb17bf97-c788-4c08-b023-8c0a1c3fb797\"},{\"content\":{\"connectorIds\":[\"RConn1\"],\"side\":\"RIGHT\"},\"type\":\"ConnectorPlacement.EquallySpacedRectSide\",\"uuid\":\"91e808db-0093-47a9-9188-f8caa3465017\"},{\"content\":{\"connectorIds\":[\"Out1\"],\"side\":\"TOP\"},\"type\":\"ConnectorPlacement.EquallySpacedRectSide\",\"uuid\":\"c8f1b688-6876-4a25-941d-460dbd5f524f\"}]},\"type\":\"ConnectorPlacement.EquallySpacedConnector\",\"uuid\":\"ee394044-67a1-441d-b622-768cddf1663c\"}],\"packageUris\":[\"http://schema.mathworks.com/mf0/Connector/R2020b\"],\"version\":\"1.0\"}"
  D4 : Subsystem
      settings: PortSchema="{\"entries\":[{\"content\":{\"sides\":[{\"content\":{\"connectorIds\":[\"LConn1\"]},\"type\":\"ConnectorPlacement.EquallySpacedRectSide\",\"uuid\":\"eb17bf97-c788-4c08-b023-8c0a1c3fb797\"},{\"content\":{\"connectorIds\":[\"RConn1\"],\"side\":\"RIGHT\"},\"type\":\"ConnectorPlacement.EquallySpacedRectSide\",\"uuid\":\"91e808db-0093-47a9-9188-f8caa3465017\"},{\"content\":{\"connectorIds\":[\"Out1\"],\"side\":\"TOP\"},\"type\":\"ConnectorPlacement.EquallySpacedRectSide\",\"uuid\":\"c8f1b688-6876-4a25-941d-460dbd5f524f\"}]},\"type\":\"ConnectorPlacement.EquallySpacedConnector\",\"uuid\":\"ee394044-67a1-441d-b622-768cddf1663c\"}],\"packageUris\":[\"http://schema.mathworks.com/mf0/Connector/R2020b\"],\"version\":\"1.0\"}"
  D5 : Subsystem
      settings: PortSchema="{\"entries\":[{\"content\":{\"sides\":[{\"content\":{\"connectorIds\":[\"LConn1\"]},\"type\":\"ConnectorPlacement.EquallySpacedRectSide\",\"uuid\":\"eb17bf97-c788-4c08-b023-8c0a1c3fb797\"},{\"content\":{\"connectorIds\":[\"RConn1\"],\"side\":\"RIGHT\"},\"type\":\"ConnectorPlacement.EquallySpacedRectSide\",\"uuid\":\"91e808db-0093-47a9-9188-f8caa3465017\"},{\"content\":{\"connectorIds\":[\"Out1\"],\"side\":\"TOP\"},\"type\":\"ConnectorPlacement.EquallySpacedRectSide\",\"uuid\":\"c8f1b688-6876-4a25-941d-460dbd5f524f\"}]},\"type\":\"ConnectorPlacement.EquallySpacedConnector\",\"uuid\":\"ee394044-67a1-441d-b622-768cddf1663c\"}],\"packageUris\":[\"http://schema.mathworks.com/mf0/Connector/R2020b\"],\"version\":\"1.0\"}"
  D6 : Subsystem
      settings: PortSchema="{\"entries\":[{\"content\":{\"sides\":[{\"content\":{\"connectorIds\":[\"LConn1\"]},\"type\":\"ConnectorPlacement.EquallySpacedRectSide\",\"uuid\":\"eb17bf97-c788-4c08-b023-8c0a1c3fb797\"},{\"content\":{\"connectorIds\":[\"RConn1\"],\"side\":\"RIGHT\"},\"type\":\"ConnectorPlacement.EquallySpacedRectSide\",\"uuid\":\"91e808db-0093-47a9-9188-f8caa3465017\"},{\"content\":{\"connectorIds\":[\"Out1\"],\"side\":\"TOP\"},\"type\":\"ConnectorPlacement.EquallySpacedRectSide\",\"uuid\":\"c8f1b688-6876-4a25-941d-460dbd5f524f\"}]},\"type\":\"ConnectorPlacement.EquallySpacedConnector\",\"uuid\":\"ee394044-67a1-441d-b622-768cddf1663c\"}],\"packageUris\":[\"http://schema.mathworks.com/mf0/Connector/R2020b\"],\"version\":\"1.0\"}"
  DC+ : PMIOPort  Side=Left
  DC- : PMIOPort  Port=2  Side=Left
  phA : PMIOPort  Port=3  Side=Right
  phB : PMIOPort  Port=4  Side=Right
  phC : PMIOPort  Port=5  Side=Right
  m_D1 : Outport
  wires:
  D1/1(m) -> m_D1/1
  connections:
  DC+/RConn1 -- D1/RConn1 -- D3/RConn1 -- D5/RConn1
  D1/LConn1 -- D2/RConn1 -- phA/RConn1
  DC-/RConn1 -- D2/LConn1 -- D6/LConn1 -- D4/LConn1
  D3/LConn1 -- D4/RConn1 -- phB/RConn1
  D5/LConn1 -- D6/RConn1 -- phC/RConn1

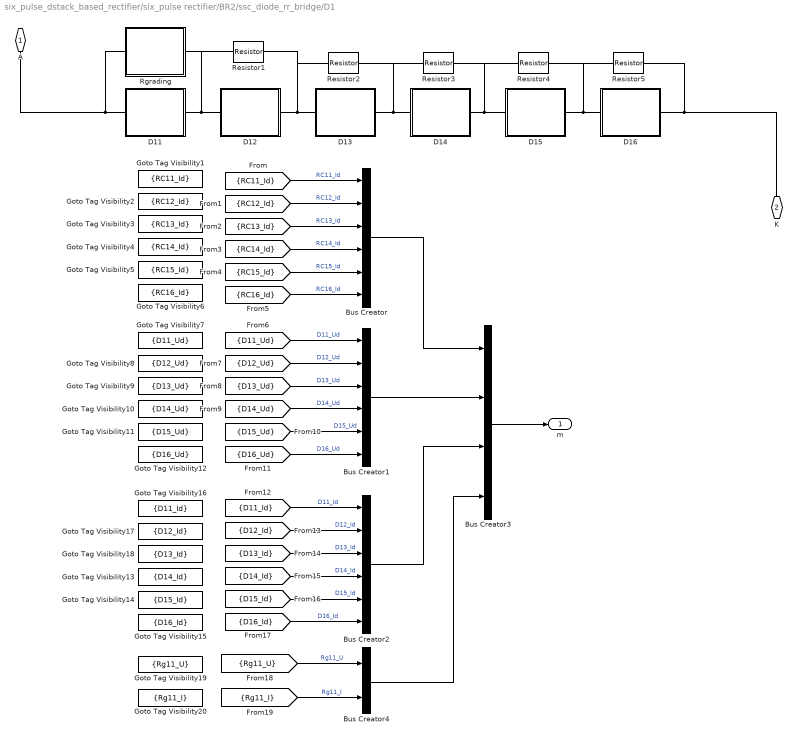
== system six_pulse_dstack_based_rectifier/six_pulse rectifier/BR2/ssc_diode_rr_bridge/D1 ==
  Bus Creator : BusCreator  Inputs=6
  Bus Creator1 : BusCreator  Inputs=6
  Bus Creator2 : BusCreator  Inputs=6
  Bus Creator3 : BusCreator  Inputs=4
  Bus Creator4 : BusCreator  Inputs=2
  D11 : Subsystem
  D12 : Subsystem
  D13 : Subsystem
  D14 : Subsystem
  D15 : Subsystem
  D16 : Subsystem
  Goto Tag Visibility1 : GotoTagVisibility  GotoTag=RC11_Id
  Goto Tag Visibility10 : GotoTagVisibility  GotoTag=D14_Ud
  Goto Tag Visibility11 : GotoTagVisibility  GotoTag=D15_Ud
  Goto Tag Visibility12 : GotoTagVisibility  GotoTag=D16_Ud
  Goto Tag Visibility13 : GotoTagVisibility  GotoTag=D14_Id
  Goto Tag Visibility14 : GotoTagVisibility  GotoTag=D15_Id
  Goto Tag Visibility15 : GotoTagVisibility  GotoTag=D16_Id
  Goto Tag Visibility16 : GotoTagVisibility  GotoTag=D11_Id
  Goto Tag Visibility17 : GotoTagVisibility  GotoTag=D12_Id
  Goto Tag Visibility18 : GotoTagVisibility  GotoTag=D13_Id
  Goto Tag Visibility19 : GotoTagVisibility  GotoTag=Rg11_U
  Goto Tag Visibility2 : GotoTagVisibility  GotoTag=RC12_Id
  Goto Tag Visibility20 : GotoTagVisibility  GotoTag=Rg11_I
  Goto Tag Visibility3 : GotoTagVisibility  GotoTag=RC13_Id
  Goto Tag Visibility4 : GotoTagVisibility  GotoTag=RC14_Id
  Goto Tag Visibility5 : GotoTagVisibility  GotoTag=RC15_Id
  Goto Tag Visibility6 : GotoTagVisibility  GotoTag=RC16_Id
  Goto Tag Visibility7 : GotoTagVisibility  GotoTag=D11_Ud
  Goto Tag Visibility8 : GotoTagVisibility  GotoTag=D12_Ud
  Goto Tag Visibility9 : GotoTagVisibility  GotoTag=D13_Ud
  Resistor{1..5} (5 alike) : fl_lib/Electrical/Electrical Elements/Resistor  R=Rgrading_m Ohm  i_specify=off  i_priority=None  i=0 A  i_nominal_specify=off  i_nominal_value=1  i_nominal_unit=A  v_specify=off  v_priority=None  v=0 V  v_nominal_specify=off  v_nominal_value=1  v_nominal_unit=V
  Rgrading : Subsystem
  A : PMIOPort  Side=Left
  K : PMIOPort  Port=2  Side=Right
  m : Outport
  wires:
  [D11_Ud] -> Bus Creator1/1  "D11_Ud"
  [D15_Ud] -> Bus Creator1/5  "D15_Ud"
  [D15_Id] -> Bus Creator2/5  "D15_Id"
  [D14_Ud] -> Bus Creator1/4  "D14_Ud"
  [D13_Id] -> Bus Creator2/3  "D13_Id"
  [D12_Ud] -> Bus Creator1/2  "D12_Ud"
  [RC12_Id] -> Bus Creator/2  "RC12_Id"
  [RC14_Id] -> Bus Creator/4  "RC14_Id"
  [D13_Ud] -> Bus Creator1/3  "D13_Ud"
  [D11_Id] -> Bus Creator2/1  "D11_Id"
  [RC16_Id] -> Bus Creator/6  "RC16_Id"
  [D14_Id] -> Bus Creator2/4  "D14_Id"
  [RC15_Id] -> Bus Creator/5  "RC15_Id"
  [RC11_Id] -> Bus Creator/1  "RC11_Id"
  [D16_Id] -> Bus Creator2/6  "D16_Id"
  [D12_Id] -> Bus Creator2/2  "D12_Id"
  [RC13_Id] -> Bus Creator/3  "RC13_Id"
  [D16_Ud] -> Bus Creator1/6  "D16_Ud"
  Bus Creator1/1 -> Bus Creator3/2
  Bus Creator/1 -> Bus Creator3/1
  Bus Creator2/1 -> Bus Creator3/3
  Bus Creator3/1 -> m/1
  [Rg11_U] -> Bus Creator4/1  "Rg11_U"
  [Rg11_I] -> Bus Creator4/2  "Rg11_I"
  Bus Creator4/1 -> Bus Creator3/4
  connections:
  D12/RConn1 -- Resistor1/RConn1 -- Resistor2/LConn1 -- D13/LConn1
  D13/RConn1 -- Resistor3/LConn1 -- Resistor2/RConn1 -- D14/LConn1
  D11/LConn1 -- Rgrading/LConn1 -- A/RConn1
  D11/RConn1 -- Rgrading/RConn1 -- Resistor1/LConn1 -- D12/LConn1
  D16/RConn1 -- Resistor5/RConn1 -- K/RConn1
  D15/RConn1 -- Resistor5/LConn1 -- Resistor4/RConn1 -- D16/LConn1
  D14/RConn1 -- Resistor3/RConn1 -- Resistor4/LConn1 -- D15/LConn1

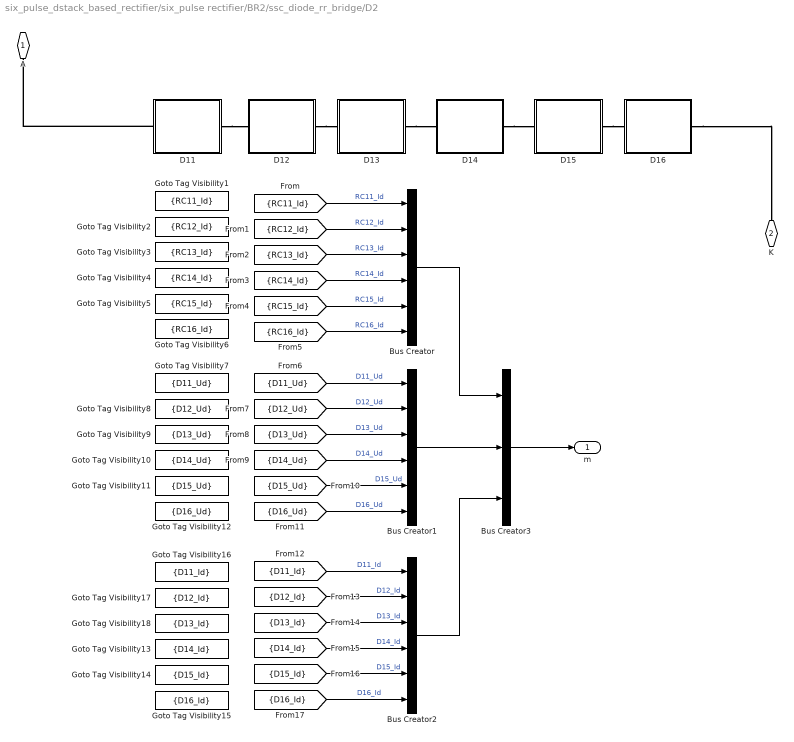
== system six_pulse_dstack_based_rectifier/six_pulse rectifier/BR2/ssc_diode_rr_bridge/D2 ==
  Bus Creator : BusCreator  Inputs=6
  Bus Creator1 : BusCreator  Inputs=6
  Bus Creator2 : BusCreator  Inputs=6
  Bus Creator3 : BusCreator  Inputs=3
  D11 : Subsystem
  D12 : Subsystem
  D13 : Subsystem
  D14 : Subsystem
  D15 : Subsystem
  D16 : Subsystem
  Goto Tag Visibility1 : GotoTagVisibility  GotoTag=RC11_Id
  Goto Tag Visibility10 : GotoTagVisibility  GotoTag=D14_Ud
  Goto Tag Visibility11 : GotoTagVisibility  GotoTag=D15_Ud
  Goto Tag Visibility12 : GotoTagVisibility  GotoTag=D16_Ud
  Goto Tag Visibility13 : GotoTagVisibility  GotoTag=D14_Id
  Goto Tag Visibility14 : GotoTagVisibility  GotoTag=D15_Id
  Goto Tag Visibility15 : GotoTagVisibility  GotoTag=D16_Id
  Goto Tag Visibility16 : GotoTagVisibility  GotoTag=D11_Id
  Goto Tag Visibility17 : GotoTagVisibility  GotoTag=D12_Id
  Goto Tag Visibility18 : GotoTagVisibility  GotoTag=D13_Id
  Goto Tag Visibility2 : GotoTagVisibility  GotoTag=RC12_Id
  Goto Tag Visibility3 : GotoTagVisibility  GotoTag=RC13_Id
  Goto Tag Visibility4 : GotoTagVisibility  GotoTag=RC14_Id
  Goto Tag Visibility5 : GotoTagVisibility  GotoTag=RC15_Id
  Goto Tag Visibility6 : GotoTagVisibility  GotoTag=RC16_Id
  Goto Tag Visibility7 : GotoTagVisibility  GotoTag=D11_Ud
  Goto Tag Visibility8 : GotoTagVisibility  GotoTag=D12_Ud
  Goto Tag Visibility9 : GotoTagVisibility  GotoTag=D13_Ud
  A : PMIOPort  Side=Left
  K : PMIOPort  Port=2  Side=Right
  m : Outport
  wires:
  Bus Creator3/1 -> m/1
  Bus Creator2/1 -> Bus Creator3/3
  Bus Creator/1 -> Bus Creator3/1
  Bus Creator1/1 -> Bus Creator3/2
  [D16_Ud] -> Bus Creator1/6  "D16_Ud"
  [RC13_Id] -> Bus Creator/3  "RC13_Id"
  [D12_Id] -> Bus Creator2/2  "D12_Id"
  [D16_Id] -> Bus Creator2/6  "D16_Id"
  [RC11_Id] -> Bus Creator/1  "RC11_Id"
  [RC15_Id] -> Bus Creator/5  "RC15_Id"
  [D14_Id] -> Bus Creator2/4  "D14_Id"
  [RC16_Id] -> Bus Creator/6  "RC16_Id"
  [D11_Id] -> Bus Creator2/1  "D11_Id"
  [D13_Ud] -> Bus Creator1/3  "D13_Ud"
  [RC14_Id] -> Bus Creator/4  "RC14_Id"
  [RC12_Id] -> Bus Creator/2  "RC12_Id"
  [D12_Ud] -> Bus Creator1/2  "D12_Ud"
  [D13_Id] -> Bus Creator2/3  "D13_Id"
  [D14_Ud] -> Bus Creator1/4  "D14_Ud"
  [D15_Id] -> Bus Creator2/5  "D15_Id"
  [D15_Ud] -> Bus Creator1/5  "D15_Ud"
  [D11_Ud] -> Bus Creator1/1  "D11_Ud"
  connections:
  D14/RConn1 -- D15/LConn1
  D15/RConn1 -- D16/LConn1
  D16/RConn1 -- K/RConn1
  D11/RConn1 -- D12/LConn1
  D11/LConn1 -- A/RConn1
  D13/RConn1 -- D14/LConn1
  D12/RConn1 -- D13/LConn1

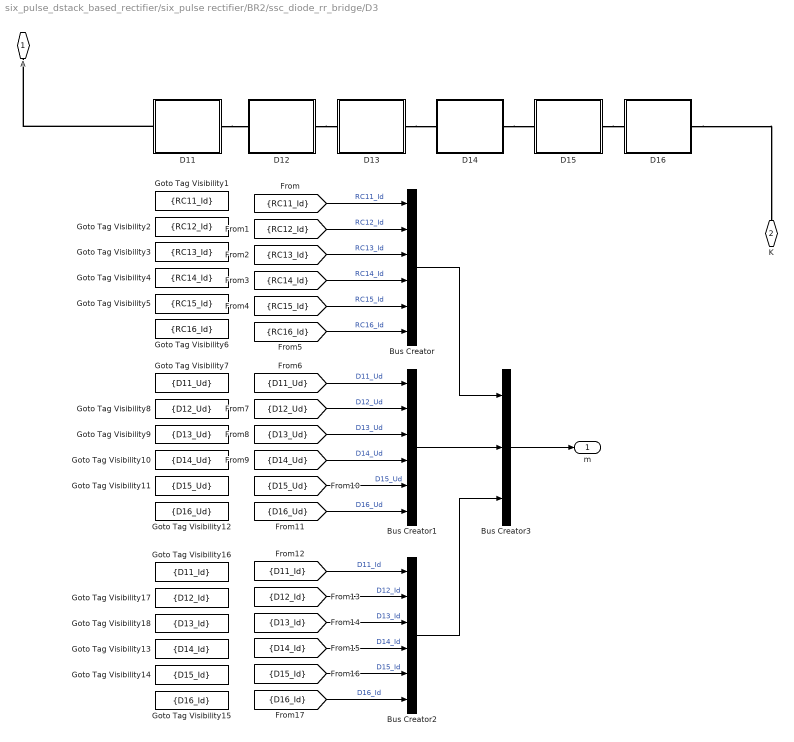
== system six_pulse_dstack_based_rectifier/six_pulse rectifier/BR2/ssc_diode_rr_bridge/D3 ==
  Bus Creator : BusCreator  Inputs=6
  Bus Creator1 : BusCreator  Inputs=6
  Bus Creator2 : BusCreator  Inputs=6
  Bus Creator3 : BusCreator  Inputs=3
  D11 : Subsystem
  D12 : Subsystem
  D13 : Subsystem
  D14 : Subsystem
  D15 : Subsystem
  D16 : Subsystem
  Goto Tag Visibility1 : GotoTagVisibility  GotoTag=RC11_Id
  Goto Tag Visibility10 : GotoTagVisibility  GotoTag=D14_Ud
  Goto Tag Visibility11 : GotoTagVisibility  GotoTag=D15_Ud
  Goto Tag Visibility12 : GotoTagVisibility  GotoTag=D16_Ud
  Goto Tag Visibility13 : GotoTagVisibility  GotoTag=D14_Id
  Goto Tag Visibility14 : GotoTagVisibility  GotoTag=D15_Id
  Goto Tag Visibility15 : GotoTagVisibility  GotoTag=D16_Id
  Goto Tag Visibility16 : GotoTagVisibility  GotoTag=D11_Id
  Goto Tag Visibility17 : GotoTagVisibility  GotoTag=D12_Id
  Goto Tag Visibility18 : GotoTagVisibility  GotoTag=D13_Id
  Goto Tag Visibility2 : GotoTagVisibility  GotoTag=RC12_Id
  Goto Tag Visibility3 : GotoTagVisibility  GotoTag=RC13_Id
  Goto Tag Visibility4 : GotoTagVisibility  GotoTag=RC14_Id
  Goto Tag Visibility5 : GotoTagVisibility  GotoTag=RC15_Id
  Goto Tag Visibility6 : GotoTagVisibility  GotoTag=RC16_Id
  Goto Tag Visibility7 : GotoTagVisibility  GotoTag=D11_Ud
  Goto Tag Visibility8 : GotoTagVisibility  GotoTag=D12_Ud
  Goto Tag Visibility9 : GotoTagVisibility  GotoTag=D13_Ud
  A : PMIOPort  Side=Left
  K : PMIOPort  Port=2  Side=Right
  m : Outport
  wires:
  Bus Creator3/1 -> m/1
  Bus Creator2/1 -> Bus Creator3/3
  Bus Creator/1 -> Bus Creator3/1
  Bus Creator1/1 -> Bus Creator3/2
  [D16_Ud] -> Bus Creator1/6  "D16_Ud"
  [RC13_Id] -> Bus Creator/3  "RC13_Id"
  [D12_Id] -> Bus Creator2/2  "D12_Id"
  [D16_Id] -> Bus Creator2/6  "D16_Id"
  [RC11_Id] -> Bus Creator/1  "RC11_Id"
  [RC15_Id] -> Bus Creator/5  "RC15_Id"
  [D14_Id] -> Bus Creator2/4  "D14_Id"
  [RC16_Id] -> Bus Creator/6  "RC16_Id"
  [D11_Id] -> Bus Creator2/1  "D11_Id"
  [D13_Ud] -> Bus Creator1/3  "D13_Ud"
  [RC14_Id] -> Bus Creator/4  "RC14_Id"
  [RC12_Id] -> Bus Creator/2  "RC12_Id"
  [D12_Ud] -> Bus Creator1/2  "D12_Ud"
  [D13_Id] -> Bus Creator2/3  "D13_Id"
  [D14_Ud] -> Bus Creator1/4  "D14_Ud"
  [D15_Id] -> Bus Creator2/5  "D15_Id"
  [D15_Ud] -> Bus Creator1/5  "D15_Ud"
  [D11_Ud] -> Bus Creator1/1  "D11_Ud"
  connections:
  D14/RConn1 -- D15/LConn1
  D15/RConn1 -- D16/LConn1
  D16/RConn1 -- K/RConn1
  D11/RConn1 -- D12/LConn1
  D11/LConn1 -- A/RConn1
  D13/RConn1 -- D14/LConn1
  D12/RConn1 -- D13/LConn1

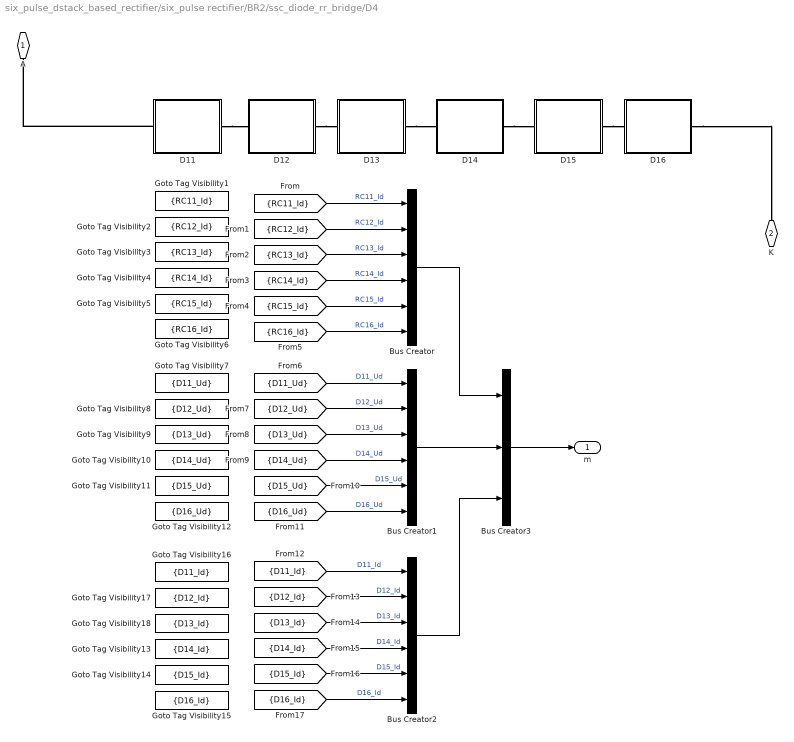
== system six_pulse_dstack_based_rectifier/six_pulse rectifier/BR2/ssc_diode_rr_bridge/D4 ==
  Bus Creator : BusCreator  Inputs=6
  Bus Creator1 : BusCreator  Inputs=6
  Bus Creator2 : BusCreator  Inputs=6
  Bus Creator3 : BusCreator  Inputs=3
  D11 : Subsystem
  D12 : Subsystem
  D13 : Subsystem
  D14 : Subsystem
  D15 : Subsystem
  D16 : Subsystem
  Goto Tag Visibility1 : GotoTagVisibility  GotoTag=RC11_Id
  Goto Tag Visibility10 : GotoTagVisibility  GotoTag=D14_Ud
  Goto Tag Visibility11 : GotoTagVisibility  GotoTag=D15_Ud
  Goto Tag Visibility12 : GotoTagVisibility  GotoTag=D16_Ud
  Goto Tag Visibility13 : GotoTagVisibility  GotoTag=D14_Id
  Goto Tag Visibility14 : GotoTagVisibility  GotoTag=D15_Id
  Goto Tag Visibility15 : GotoTagVisibility  GotoTag=D16_Id
  Goto Tag Visibility16 : GotoTagVisibility  GotoTag=D11_Id
  Goto Tag Visibility17 : GotoTagVisibility  GotoTag=D12_Id
  Goto Tag Visibility18 : GotoTagVisibility  GotoTag=D13_Id
  Goto Tag Visibility2 : GotoTagVisibility  GotoTag=RC12_Id
  Goto Tag Visibility3 : GotoTagVisibility  GotoTag=RC13_Id
  Goto Tag Visibility4 : GotoTagVisibility  GotoTag=RC14_Id
  Goto Tag Visibility5 : GotoTagVisibility  GotoTag=RC15_Id
  Goto Tag Visibility6 : GotoTagVisibility  GotoTag=RC16_Id
  Goto Tag Visibility7 : GotoTagVisibility  GotoTag=D11_Ud
  Goto Tag Visibility8 : GotoTagVisibility  GotoTag=D12_Ud
  Goto Tag Visibility9 : GotoTagVisibility  GotoTag=D13_Ud
  A : PMIOPort  Side=Left
  K : PMIOPort  Port=2  Side=Right
  m : Outport
  wires:
  [D11_Ud] -> Bus Creator1/1  "D11_Ud"
  [D15_Ud] -> Bus Creator1/5  "D15_Ud"
  [D15_Id] -> Bus Creator2/5  "D15_Id"
  [D14_Ud] -> Bus Creator1/4  "D14_Ud"
  [D13_Id] -> Bus Creator2/3  "D13_Id"
  [D12_Ud] -> Bus Creator1/2  "D12_Ud"
  [RC12_Id] -> Bus Creator/2  "RC12_Id"
  [RC14_Id] -> Bus Creator/4  "RC14_Id"
  [D13_Ud] -> Bus Creator1/3  "D13_Ud"
  [D11_Id] -> Bus Creator2/1  "D11_Id"
  [RC16_Id] -> Bus Creator/6  "RC16_Id"
  [D14_Id] -> Bus Creator2/4  "D14_Id"
  [RC15_Id] -> Bus Creator/5  "RC15_Id"
  [RC11_Id] -> Bus Creator/1  "RC11_Id"
  [D16_Id] -> Bus Creator2/6  "D16_Id"
  [D12_Id] -> Bus Creator2/2  "D12_Id"
  [RC13_Id] -> Bus Creator/3  "RC13_Id"
  [D16_Ud] -> Bus Creator1/6  "D16_Ud"
  Bus Creator1/1 -> Bus Creator3/2
  Bus Creator/1 -> Bus Creator3/1
  Bus Creator2/1 -> Bus Creator3/3
  Bus Creator3/1 -> m/1
  connections:
  D12/RConn1 -- D13/LConn1
  D13/RConn1 -- D14/LConn1
  D11/LConn1 -- A/RConn1
  D11/RConn1 -- D12/LConn1
  D16/RConn1 -- K/RConn1
  D15/RConn1 -- D16/LConn1
  D14/RConn1 -- D15/LConn1

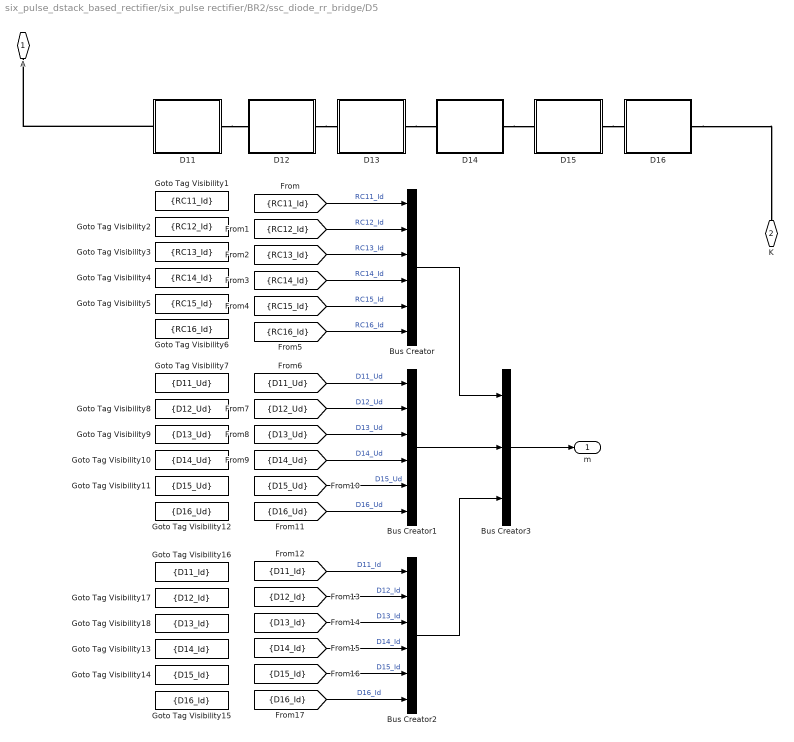
== system six_pulse_dstack_based_rectifier/six_pulse rectifier/BR2/ssc_diode_rr_bridge/D5 ==
  Bus Creator : BusCreator  Inputs=6
  Bus Creator1 : BusCreator  Inputs=6
  Bus Creator2 : BusCreator  Inputs=6
  Bus Creator3 : BusCreator  Inputs=3
  D11 : Subsystem
  D12 : Subsystem
  D13 : Subsystem
  D14 : Subsystem
  D15 : Subsystem
  D16 : Subsystem
  Goto Tag Visibility1 : GotoTagVisibility  GotoTag=RC11_Id
  Goto Tag Visibility10 : GotoTagVisibility  GotoTag=D14_Ud
  Goto Tag Visibility11 : GotoTagVisibility  GotoTag=D15_Ud
  Goto Tag Visibility12 : GotoTagVisibility  GotoTag=D16_Ud
  Goto Tag Visibility13 : GotoTagVisibility  GotoTag=D14_Id
  Goto Tag Visibility14 : GotoTagVisibility  GotoTag=D15_Id
  Goto Tag Visibility15 : GotoTagVisibility  GotoTag=D16_Id
  Goto Tag Visibility16 : GotoTagVisibility  GotoTag=D11_Id
  Goto Tag Visibility17 : GotoTagVisibility  GotoTag=D12_Id
  Goto Tag Visibility18 : GotoTagVisibility  GotoTag=D13_Id
  Goto Tag Visibility2 : GotoTagVisibility  GotoTag=RC12_Id
  Goto Tag Visibility3 : GotoTagVisibility  GotoTag=RC13_Id
  Goto Tag Visibility4 : GotoTagVisibility  GotoTag=RC14_Id
  Goto Tag Visibility5 : GotoTagVisibility  GotoTag=RC15_Id
  Goto Tag Visibility6 : GotoTagVisibility  GotoTag=RC16_Id
  Goto Tag Visibility7 : GotoTagVisibility  GotoTag=D11_Ud
  Goto Tag Visibility8 : GotoTagVisibility  GotoTag=D12_Ud
  Goto Tag Visibility9 : GotoTagVisibility  GotoTag=D13_Ud
  A : PMIOPort  Side=Left
  K : PMIOPort  Port=2  Side=Right
  m : Outport
  wires:
  [D11_Ud] -> Bus Creator1/1  "D11_Ud"
  [D15_Ud] -> Bus Creator1/5  "D15_Ud"
  [D15_Id] -> Bus Creator2/5  "D15_Id"
  [D14_Ud] -> Bus Creator1/4  "D14_Ud"
  [D13_Id] -> Bus Creator2/3  "D13_Id"
  [D12_Ud] -> Bus Creator1/2  "D12_Ud"
  [RC12_Id] -> Bus Creator/2  "RC12_Id"
  [RC14_Id] -> Bus Creator/4  "RC14_Id"
  [D13_Ud] -> Bus Creator1/3  "D13_Ud"
  [D11_Id] -> Bus Creator2/1  "D11_Id"
  [RC16_Id] -> Bus Creator/6  "RC16_Id"
  [D14_Id] -> Bus Creator2/4  "D14_Id"
  [RC15_Id] -> Bus Creator/5  "RC15_Id"
  [RC11_Id] -> Bus Creator/1  "RC11_Id"
  [D16_Id] -> Bus Creator2/6  "D16_Id"
  [D12_Id] -> Bus Creator2/2  "D12_Id"
  [RC13_Id] -> Bus Creator/3  "RC13_Id"
  [D16_Ud] -> Bus Creator1/6  "D16_Ud"
  Bus Creator1/1 -> Bus Creator3/2
  Bus Creator/1 -> Bus Creator3/1
  Bus Creator2/1 -> Bus Creator3/3
  Bus Creator3/1 -> m/1
  connections:
  D12/RConn1 -- D13/LConn1
  D13/RConn1 -- D14/LConn1
  D11/LConn1 -- A/RConn1
  D11/RConn1 -- D12/LConn1
  D16/RConn1 -- K/RConn1
  D15/RConn1 -- D16/LConn1
  D14/RConn1 -- D15/LConn1

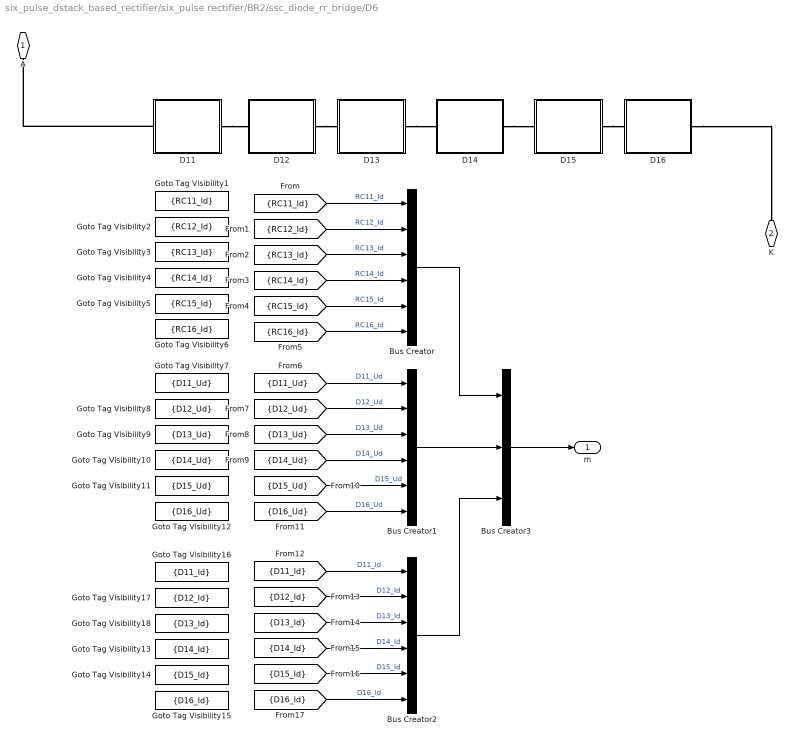
== system six_pulse_dstack_based_rectifier/six_pulse rectifier/BR2/ssc_diode_rr_bridge/D6 ==
  Bus Creator : BusCreator  Inputs=6
  Bus Creator1 : BusCreator  Inputs=6
  Bus Creator2 : BusCreator  Inputs=6
  Bus Creator3 : BusCreator  Inputs=3
  D11 : Subsystem
  D12 : Subsystem
  D13 : Subsystem
  D14 : Subsystem
  D15 : Subsystem
  D16 : Subsystem
  Goto Tag Visibility1 : GotoTagVisibility  GotoTag=RC11_Id
  Goto Tag Visibility10 : GotoTagVisibility  GotoTag=D14_Ud
  Goto Tag Visibility11 : GotoTagVisibility  GotoTag=D15_Ud
  Goto Tag Visibility12 : GotoTagVisibility  GotoTag=D16_Ud
  Goto Tag Visibility13 : GotoTagVisibility  GotoTag=D14_Id
  Goto Tag Visibility14 : GotoTagVisibility  GotoTag=D15_Id
  Goto Tag Visibility15 : GotoTagVisibility  GotoTag=D16_Id
  Goto Tag Visibility16 : GotoTagVisibility  GotoTag=D11_Id
  Goto Tag Visibility17 : GotoTagVisibility  GotoTag=D12_Id
  Goto Tag Visibility18 : GotoTagVisibility  GotoTag=D13_Id
  Goto Tag Visibility2 : GotoTagVisibility  GotoTag=RC12_Id
  Goto Tag Visibility3 : GotoTagVisibility  GotoTag=RC13_Id
  Goto Tag Visibility4 : GotoTagVisibility  GotoTag=RC14_Id
  Goto Tag Visibility5 : GotoTagVisibility  GotoTag=RC15_Id
  Goto Tag Visibility6 : GotoTagVisibility  GotoTag=RC16_Id
  Goto Tag Visibility7 : GotoTagVisibility  GotoTag=D11_Ud
  Goto Tag Visibility8 : GotoTagVisibility  GotoTag=D12_Ud
  Goto Tag Visibility9 : GotoTagVisibility  GotoTag=D13_Ud
  A : PMIOPort  Side=Left
  K : PMIOPort  Port=2  Side=Right
  m : Outport
  wires:
  Bus Creator3/1 -> m/1
  Bus Creator2/1 -> Bus Creator3/3
  Bus Creator/1 -> Bus Creator3/1
  Bus Creator1/1 -> Bus Creator3/2
  [D16_Ud] -> Bus Creator1/6  "D16_Ud"
  [RC13_Id] -> Bus Creator/3  "RC13_Id"
  [D12_Id] -> Bus Creator2/2  "D12_Id"
  [D16_Id] -> Bus Creator2/6  "D16_Id"
  [RC11_Id] -> Bus Creator/1  "RC11_Id"
  [RC15_Id] -> Bus Creator/5  "RC15_Id"
  [D14_Id] -> Bus Creator2/4  "D14_Id"
  [RC16_Id] -> Bus Creator/6  "RC16_Id"
  [D11_Id] -> Bus Creator2/1  "D11_Id"
  [D13_Ud] -> Bus Creator1/3  "D13_Ud"
  [RC14_Id] -> Bus Creator/4  "RC14_Id"
  [RC12_Id] -> Bus Creator/2  "RC12_Id"
  [D12_Ud] -> Bus Creator1/2  "D12_Ud"
  [D13_Id] -> Bus Creator2/3  "D13_Id"
  [D14_Ud] -> Bus Creator1/4  "D14_Ud"
  [D15_Id] -> Bus Creator2/5  "D15_Id"
  [D15_Ud] -> Bus Creator1/5  "D15_Ud"
  [D11_Ud] -> Bus Creator1/1  "D11_Ud"
  connections:
  D14/RConn1 -- D15/LConn1
  D15/RConn1 -- D16/LConn1
  D16/RConn1 -- K/RConn1
  D11/RConn1 -- D12/LConn1
  D11/LConn1 -- A/RConn1
  D13/RConn1 -- D14/LConn1
  D12/RConn1 -- D13/LConn1

== system six_pulse_dstack_based_rectifier/six_pulse rectifier/BR2/ssc_diode_rr_bridge/D1/D11 ==
  D11 : Subsystem
      settings: PortSchema="{\"entries\":[{\"content\":{\"sides\":[{\"content\":{},\"type\":\"ConnectorPlacement.EquallySpacedRectSide\",\"uuid\":\"7269b907-ab9b-4481-ac18-a8dd984c3818\"},{\"content\":{\"side\":\"RIGHT\"},\"type\":\"ConnectorPlacement.EquallySpacedRectSide\",\"uuid\":\"8dceca02-62a3-4342-b624-c7d4418298d0\"},{\"content\":{\"connectorIds\":[\"LConn1\"],\"side\":\"TOP\"},\"type\":\"ConnectorPlacement.EquallySpacedRectSide\",\"uuid\":\"a3401fa4-31f5-4c91-8a09-9f2730c54d6f\"},{\"content\":{\"connectorIds\":[\"RConn1\"],\"side\":\"BOTTOM\"},\"type\":\"ConnectorPlacement.EquallySpacedRectSide\",\"uuid\":\"ec3e6ca2-4822-4b63-8ee1-1049d14efe1d\"}]},\"type\":\"ConnectorPlacement.EquallySpacedConnector\",\"uuid\":\"06f44f8b-bef4-44e1-af36-23832e4d595a\"}],\"packageUris\":[\"http://schema.mathworks.com/mf0/Connector/R2020b\"],\"version\":\"1.0\"}"
  K : PMIOPort  Side=Right
  A : PMIOPort  Port=2  Side=Left
  connections:
  D11/LConn1 -- K/RConn1
  A/RConn1 -- D11/RConn1
